simulink model "sm_car"  (R2025a)
settings: Solver=ode23t  StartTime=0.0  StopTime=400  MaxStep=0.4  RelTol=1e-3  AbsTol=1e-3  EnableMultiTasking=on
PreLoadFcn:
  | % Due to usability issue in Repeating Sequence block
  | warning('off','Simulink:Masking:Invalid');
  | 
  | % Eliminate unnecessary warnings in inactive variants
  | % Warnings generated only if you click through inactive variant
  | warning('off','MATLAB:nonExistentField');
  | warning('off','Simulink:Parameters:BlkParamUndefined');
PostLoadFcn:
  | set_param([bdroot '/Vehicle'],'popup_trailer','Off')
  | warning('off','sm:sli:setup:compile:LocalSolverNotSupported')
  | %sm_car_config_maneuver(bdroot,'WOT Braking');
  | sm_car_config_vehicle(bdroot,'false');
  | sm_car_config_logging(bdroot);
InitFcn:
  | sm_car_config_camera;
  | Vehicle = sm_car_vehcfg_checkConfig(Vehicle);
  | sm_car_check_tire_model(bdroot);
StartFcn:
  | tic;
StopFcn:
  | Elapsed_Sim_Time = toc;
  | % disp(['Elapsed Sim Time = ' num2str(Elapsed_Sim_Time)]);
undefined symbols (not defined in the file): Axle1D, AxleIn, Camera, Control, Driver, Free, Init, Maneuver, Pedal, RaceFix, RaceSpin, Scene, ShaftL1, ShaftL2, ShaftR1, ShaftR2, Soft, Stiff, Visual, X, xy_data_car_side, Y, Z
libraries: sm_lib x1546, nesl_utility x528, fl_lib x480, SimscapeFluids_lib x61, sdl_lib x49, simulink x29, ee_lib x7, simulink_extras x6, Linkage_Systems x4, Tire_1x2x x4, AntiRollBar_Systems x2, Linkage_Decoupled x2
(part 79 of 79)

== matlab function sm_car/Driver/Closed Loop/Driver/Lateral Driver/Stanley/Stanley Driver ==
  data: referencePose input; steeringAngle output; currentPose input; v_x input; direction input; L_AXLE_DIST input; MAX_STEERING_ANGLE_DEG input; K_cte_forward input; K_cte_reverse input
function steeringAngle = lateralDrivingController(referencePose, currentPose, v_x, direction, L_AXLE_DIST, MAX_STEERING_ANGLE_DEG, K_cte_forward, K_cte_reverse)
%#codegen % Directive for MATLAB Coder

% lateralDrivingController Implements Stanley method for lateral control.
% Supports forward and reverse driving.
% Based on Hoffmann et al. (2007), "Autonomous Automobile Trajectory Tracking for Off-Road Driving"
%
% Inputs:
%   referencePose: [x_ref, y_ref, yaw_ref] (1x3 double vector)
%       x_ref: Reference x-coordinate (m) on the path (closest point)
%       y_ref: Reference y-coordinate (m) on the path (closest point)
%       yaw_ref: Reference yaw angle (rad) of the path tangent at (x_ref, y_ref)
%   currentPose: [x_curr, y_curr, yaw_curr] (1x3 double vector)
%       x_curr: Current x-coordinate (m) of the vehicle's reference point (e.g., rear axle center)
%       y_curr: Current y-coordinate (m) of the vehicle's reference point
%       yaw_curr: Current yaw angle (rad) of the vehicle
%   v_x: Current longitudinal velocity (m/s) of the vehicle.
%        Positive for forward, can be negative for reverse (though 'direction' input is primary).
%   direction: Driving direction (+1 for forward, -1 for reverse). (scalar double)
%
% Output:
%   steeringAngle: Calculated steering angle (rad) of the front wheels.
%                  Positive for left turn, negative for right turn.

% --- Controller Parameters (Tunable) ---
% K_cte = Driver.Lateral.NForward.Value  ;  % Cross-track error gain (Stanley gain 'k'). Adjust based on vehicle.
              % Typical values: 0.3 to 1.0. Higher values lead to more aggressive correction.

% L_AXLE_DIST = Driver.Lateral.xWheelbase.Value; % Distance from the vehicle's reference point (currentPose)
                                                % to the front axle (m). If currentPose is rear axle, this is wheelbase.

SOFTENING_CONSTANT_V = 0.1; % Small constant (epsilon) to prevent division by zero or
                            % overly aggressive steering at very low speeds (m/s).
                            % Should be small, e.g., 0.01 to 0.5.

MAX_STEERING_ANGLE = MAX_STEERING_ANGLE_DEG * (pi/180)  ; % Maximum steering angle (radians)
% MIN_VELOCITY_FOR_CONTROL is implicitly handled by SOFTENING_CONSTANT_V and using abs(v_x)

% --- Input Validation / Pre-processing (Basic) ---
referencePose = referencePose(:)';
currentPose = currentPose(:)';

% --- Extract Pose Components ---
x_vehicle_ref_pt   = currentPose(1); % x of vehicle's defined reference point (e.g., rear axle)
y_vehicle_ref_pt   = currentPose(2); % y of vehicle's defined reference point
yaw_vehicle        = currentPose(3); % Vehicle's current yaw angle

x_path   = referencePose(1); % x of closest point on path
y_path   = referencePose(2); % y of closest point on path
yaw_path = referencePose(3); % Tangent angle of path at (x_path, y_path)

% --- 1. Calculate Front Axle Position ---
% Stanley controller operates on the error at the front axle.
% (x_fa, y_fa) in the paper's notation.
x_front_axle = x_vehicle_ref_pt + L_AXLE_DIST * cos(yaw_vehicle);
y_front_axle = y_vehicle_ref_pt + L_AXLE_DIST * sin(yaw_vehicle);

% --- 2. Calculate Heading Error (phi_e in paper, psi_e here) ---
% Difference between path yaw and vehicle yaw.
% phi_e = yaw_path - yaw_vehicle
heading_error_raw = yaw_path - yaw_vehicle;
psi_e = atan2(sin(heading_error_raw), cos(heading_error_raw)); % Normalize to [-pi, pi]

% --- 3. Calculate Cross-Track Error (e_fa) at the Front Axle ---
% As per Hoffmann et al. (2007), e_fa is positive if the path is to the
% RIGHT of the vehicle's front axle.
% e_fa = (x_front_axle - x_path) * sin(yaw_path) - (y_front_axle - y_path) * cos(yaw_path);
%
% Let dx_fa = x_front_axle - x_path
% Let dy_fa = y_front_axle - y_path
% The vector from path point to front axle is [dx_fa, dy_fa].
% The path tangent vector is [cos(yaw_path), sin(yaw_path)].
% The path normal vector pointing to the RIGHT of the path is [sin(yaw_path), -cos(yaw_path)].
% e_fa is the projection of [dx_fa, dy_fa] onto this normal vector.
dx_fa = x_front_axle - x_path;
dy_fa = y_front_axle - y_path;

e_fa = dx_fa * sin(yaw_path) - dy_fa * cos(yaw_path);
% Note on sign:
% If front axle is to the LEFT of path, e_fa will be NEGATIVE.
% If front axle is to the RIGHT of path, e_fa will be POSITIVE.

% --- 4. Calculate Steering Angle Components ---

% Cross-track error steering component (delta_e in paper's combined formula)
% delta_e = arctan(k * e_fa / (v_x + softening_constant))
% Use absolute velocity for the denominator to handle forward/reverse consistently
% and add softening constant.
% The paper's v_x in the denominator implies speed magnitude.
effective_velocity_for_atan = abs(v_x) + SOFTENING_CONSTANT_V;

if direction == 1
    delta_cte = atan2(K_cte_forward *  e_fa, effective_velocity_for_atan);
else % if direction == -1
    delta_cte = atan2(K_cte_reverse * -e_fa, effective_velocity_for_atan);
end

% --- 5. Combine Steering Components (Stanley Law) with Directionality ---
% Standard Stanley Law for forward motion:
% steeringAngleUnsaturated = psi_e + delta_cte;
%
% For REVERSE motion (direction = -1):
% The overall steering command needs to be inverted because the vehicle steers
% from the "rear" effectively.
%   - If heading error (psi_e) is positive (path to the left of vehicle yaw),
%     for forward, steer left. For reverse, to make rear go left, steer front right.
%   - If cross-track error (e_fa negative -> front axle left of path),
%     for forward, delta_cte is negative (steer right). For reverse, to make
%     front axle move right (and thus vehicle move right towards path), steer front left.
%
% So, the entire calculated "forward" steering command is multiplied by 'direction'.
steeringAngleUnsaturated = direction * (psi_e + delta_cte);

% --- 6. Saturate Steering Angle ---
if steeringAngleUnsaturated > MAX_STEERING_ANGLE
    steeringAngle = MAX_STEERING_ANGLE;
elseif steeringAngleUnsaturated < -MAX_STEERING_ANGLE
    steeringAngle = -MAX_STEERING_ANGLE;
else
    steeringAngle = steeringAngleUnsaturated;
end

% --- (Optional) Debugging Outputs ---
% coder.extrinsic('fprintf'); % Allow fprintf for debugging during simulation
% fprintf('Dir: %d, YawVeh: %.2f, YawPath: %.2f, psi_e: %.2f\n', direction, yaw_vehicle, yaw_path, psi_e);
% fprintf('x_fa: %.2f, y_fa: %.2f, e_fa: %.2f\n', x_front_axle, y_front_axle, e_fa);
% fprintf('v_x: %.2f, eff_v: %.2f, delta_cte: %.2f\n', v_x, effective_velocity_for_atan, delta_cte);
% fprintf('UnsatSteer: %.3f, Steering cmd: %.3f\n', steeringAngleUnsaturated, steeringAngle);

end

== matlab function sm_car/Driver/Closed Loop/Driver/Longitudinal Driver/Longitudinal Driver ==
  settings: sampleTime=0.1
  data: pp_preview_dist_pts input; AccelCmd output; pp_preview_speed_pts input; ad_vehicle input; current_vx input; dir input; current_slope_rad input; SPEED_LOOKAHEAD_TIME input; VEHICLE_MASS_KG input; GRAVITY_MPS2 input; C_ROLLING_RESISTANCE_COEFF input; C_AERO_DRAG_COEFF input; MAX_NET_DRIVING_FORCE_N input; MAX_NET_BRAKING_FORCE_N input; KP_SPEED input; KI_SPEED input; MAX_ACCEL_MPS2 input; MAX_DECEL_MPS2 input; integral_error_input input; DecelCmd output; v_error_out output
function [AccelCmd, DecelCmd, v_error_out] = longitudinalSpeedController(...
    pp_preview_dist_pts, ...     % Preview segment: cumulative distances (m)
    pp_preview_speed_pts, ...    % Preview segment: target speeds (m/s)
    ad_vehicle, ...              % Current distance of vehicle along path (m)
    current_vx, ...              % Vehicle's current longitudinal velocity (m/s)
    dir, current_slope_rad, ...       % Current road slope/gradient (radians, positive for uphill)    
    SPEED_LOOKAHEAD_TIME, ...    % Lookahead time (s)
    VEHICLE_MASS_KG, ...         % Vehicle mass (kg)
    GRAVITY_MPS2, ...            % Acceleration due to gravity (m/s^2)
    C_ROLLING_RESISTANCE_COEFF, ...    % Rolling resistance coefficient
    C_AERO_DRAG_COEFF, ...             % Aerodynamic drag coefficient (0.5 * rho * A * Cd)
    MAX_NET_DRIVING_FORCE_N, ... % Max net driving force at wheels (engine limit - min resistances)
    MAX_NET_BRAKING_FORCE_N, ... % Max net braking force at wheels (brake limit + engine braking if modeled)
    KP_SPEED, ...                % Proportional gain for speed PI controller (normalized value using max_force_contribution)
    KI_SPEED, ...                % Integral gain for speed PI controller (normalized value using max_force_contribution)
    MAX_ACCEL_MPS2, ...          % Max desired acceleration (for feedforward and limiting)
    MAX_DECEL_MPS2, ...          % Max desired deceleration (negative value, e.g., -5 m/s^2)
    integral_error_input)...     % Externally integrated speed error (m) %#ok<INUSD>

%#codegen

% longitudinalSpeedController Implements a PI controller with feedforward
% for velocity tracking, outputting acceleration/deceleration commands and speed error.
% Designed for continuous-time simulation with external error integration.
%
% Outputs:
%   AccelCmd: Normalized acceleration command [0, 1]
%   DecelCmd: Normalized deceleration command [0, 1] (positive value)
%   v_error_out: Current speed error (v_target - v_actual) (m/s)

%  1. Determine Target Velocity and Desired Acceleration from Preview 
lookahead_dist_for_speed = current_vx * SPEED_LOOKAHEAD_TIME;
target_cumulative_dist_for_speed = ad_vehicle + lookahead_dist_for_speed;

num_preview_pts = length(pp_preview_dist_pts);
v_target_at_lookahead = current_vx; % Default to current speed if no preview

thisSeg = 0;
pp_preview_speed_pts = pp_preview_speed_pts*dir;
if num_preview_pts > 0
    if target_cumulative_dist_for_speed <= pp_preview_dist_pts(1)
        v_target_at_lookahead = pp_preview_speed_pts(1);
    elseif target_cumulative_dist_for_speed >= pp_preview_dist_pts(end)
        v_target_at_lookahead = pp_preview_speed_pts(end);
    else
        % Interpolate to find target speed at lookahead distance
        % (Using existing interpolation logic, could be replaced with interp1)
        for n = 1:(num_preview_pts-1)
            if target_cumulative_dist_for_speed >= pp_preview_dist_pts(n) && ...
               target_cumulative_dist_for_speed < pp_preview_dist_pts(n+1)
                % Ensure denominator is not zero for robust interpolation
                fraction_denom = pp_preview_dist_pts(n+1) - pp_preview_dist_pts(n);
                if fraction_denom > 1e-6 % Avoid division by zero if points are coincident
                    fraction = (target_cumulative_dist_for_speed - pp_preview_dist_pts(n)) / fraction_denom;
                    v_target_at_lookahead = pp_preview_speed_pts(n) + ...
                                       fraction * (pp_preview_speed_pts(n+1) - pp_preview_speed_pts(n));
                else % Points are too close, take the speed of the first point of the pair
                    v_target_at_lookahead = pp_preview_speed_pts(n);
                end
                break; 
            end
            thisSeg = n;
        end
         % Handle case where loop finishes, and target is beyond the last segment start but not caught by pp_preview_dist_pts(end)
         if (thisSeg == (num_preview_pts-1)) && (target_cumulative_dist_for_speed >= pp_preview_dist_pts(end))
            v_target_at_lookahead = pp_preview_speed_pts(end);
         end
    end
end

% Determine desired feedforward acceleration based on a short lookahead on the preview path
idx_current_on_preview = 1;
for n = 1:num_preview_pts
    if ad_vehicle >= pp_preview_dist_pts(n)
        idx_current_on_preview = n;
    else
        break;
    end
end

idx_future_on_preview = idx_current_on_preview;
dist_for_accel_calc = current_vx * 0.1; % Short distance ahead for accel calculation (e.g., 0.2s at current speed)
for n = idx_current_on_preview:num_preview_pts
    if (pp_preview_dist_pts(n) - ad_vehicle) >= dist_for_accel_calc
        idx_future_on_preview = n;
        break;
    end
    if n == num_preview_pts % Reached end of preview
        idx_future_on_preview = num_preview_pts;
    end
end

a_desired_feedforward = 0.0; % Initialize
if idx_future_on_preview > idx_current_on_preview && num_preview_pts > 1
    delta_v = pp_preview_speed_pts(idx_future_on_preview) - pp_preview_speed_pts(idx_current_on_preview);
    delta_d = pp_preview_dist_pts(idx_future_on_preview) - pp_preview_dist_pts(idx_current_on_preview);

    if delta_d > 1e-3 % Ensure segment has some physical length
        v_avg_segment = (pp_preview_speed_pts(idx_future_on_preview) + pp_preview_speed_pts(idx_current_on_preview)) / 2.0;
        
        denominator_v_avg = max(0.1, abs(v_avg_segment)); % Robust denominator for delta_t
        delta_t_segment = delta_d / denominator_v_avg;

        MIN_SEGMENT_TIME_FOR_FF = 1e-3; % Min segment time (s) for a meaningful FF accel calculation
        if delta_t_segment > MIN_SEGMENT_TIME_FOR_FF
            a_desired_feedforward = delta_v / delta_t_segment;
        end
    end
end

if(dir>0)
a_desired_feedforward = max(MAX_DECEL_MPS2, min(a_desired_feedforward, MAX_ACCEL_MPS2)); % Clamp
else
a_desired_feedforward = max(-MAX_ACCEL_MPS2, min(a_desired_feedforward, -MAX_DECEL_MPS2)); % Clamp
end


%  2. Calculate Feedforward Force using Simple Vehicle Model 
F_rolling = C_ROLLING_RESISTANCE_COEFF * VEHICLE_MASS_KG * GRAVITY_MPS2 * cos(current_slope_rad);
F_aero    = C_AERO_DRAG_COEFF * current_vx^2;
F_gravity = VEHICLE_MASS_KG * GRAVITY_MPS2 * sin(current_slope_rad);
F_resist = F_rolling + F_aero + F_gravity;
F_wheels_feedforward = VEHICLE_MASS_KG * a_desired_feedforward - F_resist;

%  3. PI Feedback Controller 
v_error = v_target_at_lookahead - current_vx;
P_term = KP_SPEED * v_error;

% I_term uses externally integrated error
I_term_unclamped = KI_SPEED * integral_error_input;

% Anti-windup: Clamp the force contribution of the I-term
% This assumes integral_error_input is the raw integral.
% The clamping limits the *effect* of very large integrated errors.
max_force_contribution = max(MAX_NET_DRIVING_FORCE_N, MAX_NET_BRAKING_FORCE_N);
I_term = max(-max_force_contribution, min(I_term_unclamped, max_force_contribution));

% Change the PI control to physical values
F_pi_correction = max_force_contribution * (P_term + I_term);

%  4. Combine Feedforward and Feedback 
F_total_desired_at_wheels = F_wheels_feedforward + F_pi_correction;

%  5. Convert Total Desired Force to Normalized Actuation Command [-1, +1] 
actuationCmd = 0.0; % This is the command before any (external) rate limiting

if F_total_desired_at_wheels > 0 % Needs net driving force
    if MAX_NET_DRIVING_FORCE_N > 1e-6 
        actuationCmd = F_total_desired_at_wheels / MAX_NET_DRIVING_FORCE_N;
    end
    actuationCmd = max(0, min(actuationCmd, 1.0)); % Clamp to [0, 1]

elseif F_total_desired_at_wheels < 0 % Needs net braking force
    if MAX_NET_BRAKING_FORCE_N > 1e-6
        actuationCmd = F_total_desired_at_wheels / MAX_NET_BRAKING_FORCE_N; % Will be negative
    end
    actuationCmd = max(-1.0, min(actuationCmd, 0)); % Clamp to [-1, 0]
else
    actuationCmd = 0.0; % Coast
end

% Ensure strictly within [-1, 1] (already handled by clamping in step 5)
% actuationCmd = max(-1.0, min(actuationCmd, 1.0));

% Outputs
if actuationCmd >= 0
    AccelCmd = actuationCmd;
    DecelCmd = 0.0;
else
    AccelCmd = 0.0;
    DecelCmd = -actuationCmd; % DecelCmd is positive, range [0, 1]
end

v_error_out = v_error; % Output current speed error for external integration

%  Debugging Outputs (Optional, ensure coder.extrinsic if used in codegen)
% coder.extrinsic('fprintf');
% fprintf('Vcurr: %.2f, Vtgt_LH: %.2f, Verr: %.2f\n', current_vx, v_target_at_lookahead, v_error);
% fprintf('Ades_FF: %.2f, F_wheels_FF: %.1f, F_PI: %.1f, F_total_des: %.1f\n', ...
%         a_desired_feedforward, F_wheels_feedforward, F_pi_correction, F_total_desired_at_wheels);
% fprintf('CmdUnrated: %.3f\n', actuationCmd);

end

== matlab function sm_car/Driver/Closed Loop/Maneuver/MATLAB Function ==
  data: ref_z output; ad output; ref_x output; ref_y output; ref_ayaw output; vTarget output; ld output; cp output; simres output; pp_preview_x_pts output; pp_preview_y_pts output; pp_preview_yaw_pts output; pp_preview_dist_pts output; pp_preview_speed_pts output; idx_ptMin output; p input; q input; posx input; posy input; posz input; speed input; xywin input; yaw input; dist input; pd input; maxld input; minSpd input; speedGain input; idx_ptMin_prev input; nPreviewPoints parameter
function [ref_z,ad,ref_x,ref_y,ref_ayaw,vTarget,ld,cp,  simres, ...
          pp_preview_x_pts, pp_preview_y_pts, pp_preview_yaw_pts, pp_preview_dist_pts, pp_preview_speed_pts,idx_ptMin] = ...
          getPoseCurRef(p,q,posx,posy,posz,speed,xywin,yaw,dist,pd, ...
                        maxld, minSpd, speedGain, idx_ptMin_prev, nPreviewPoints)

% This function determines the target pose for the vehicle.  It
% interpolates within the provided trajectory to determine the target
% x-y position, yaw angle, and speed. The targets are defined with respect
% to distance along the target trajectory.  The first portion of the
% function determines the distance along the trajectory that the vehicle
% has traveled (ad).  Once that is found, the function interpolates to find
% the target pose at the preview distance (ad+pd).

npts = length(posx);

% Look for nearest point in a window near last evaluation
% Obtain window
if (idx_ptMin_prev == -1)
    % For first evaluation, use entire list of points
    ptlist = 1:npts;
elseif((idx_ptMin_prev-xywin)<1)
    % Window overlaps at lower end: take points from upper end
    win2 = (npts+idx_ptMin_prev-xywin):1:npts;
    win1 = 1:(idx_ptMin_prev+xywin);
    ptlist = [win1 win2];
elseif((idx_ptMin_prev+xywin)>npts)
    % Window overlaps at upper end: take points from lower end
    win2 = (idx_ptMin_prev-xywin):1:npts;
    win1 = 1:(idx_ptMin_prev+xywin-npts);
    ptlist = [win1 win2];
else
    % No overlap: use window
    ptlist = (idx_ptMin_prev-xywin):1:(idx_ptMin_prev+xywin);
end

% Find closest supplied trajectory point to current car position
distances = hypot(p(1) - posx,p(2) - posy);
distances_srch = distances(ptlist);
[~, idx_ptlist] = min(distances_srch);
idx_ptMin = ptlist(idx_ptlist);

%% Identify two trajectory points ahead of and behind closest supplied point
% A, B, C (closest), D, E
idx_ptC = idx_ptMin;
idx_ptA = idx_ptMin-2;
idx_ptB = idx_ptMin-1;
idx_ptD = idx_ptMin+1;
idx_ptE = idx_ptMin+2;

% If we are at end of trajectory, wrap point index
if (idx_ptA<=0),   idx_ptA = idx_ptA+npts; end
if (idx_ptB<=0),   idx_ptB = idx_ptB+npts; end
if (idx_ptD>npts), idx_ptD = idx_ptD-npts; end
if (idx_ptE>npts), idx_ptE = idx_ptE-npts; end

% Extract trajectory point x-y locations
ptA = [posx(idx_ptA); posy(idx_ptA)];
ptB = [posx(idx_ptB); posy(idx_ptB)];
ptC = [posx(idx_ptC); posy(idx_ptC)];
ptD = [posx(idx_ptD); posy(idx_ptD)];
ptE = [posx(idx_ptE); posy(idx_ptE)];

%% Find line separating trajectory segments BC, CD
% Find angle of line connecting BD
qBD = atan2(ptD(2)-ptB(2),ptD(1)-ptB(1));

% Angle of line separating BC, CD is normal to that line
qC  = qBD+pi/2;

%% Determine if we are nearest to trajectory segment BC or BD
% Check if vehicle location and point B on same side of line
% separating segments BC and BD
segBC = arePointsOnSameSide(ptC(1), ptC(2), tan(qC), p(1), p(2), ptB(1), ptB(2));

%% Find vehicle line segment 
% Segment is parallel to closest trajectory segment on which vehicle lies
if(segBC)
   % Use segment BC
   % Line dividing segments AB and BC is normal to line AC 
   qR = atan2(ptC(2)-ptA(2),ptC(1)-ptA(1))+pi/2;
   % Line dividing segments BC and CD has already been found 
   qF = qC;

   ptR = ptB;  % Rear point of segment is point B
   ptF = ptC;  % Front point of segment is point C

   % Angle of vehicle line segment is same as angle of segment BC
   qV = atan2(ptC(2)-ptB(2),ptC(1)-ptB(1));
    % Distance along trajectory to rear of segment
   distR    = dist(idx_ptB);
else
   % Use segment CD
   % Line dividing segments BC and CD has already been found 
   qR = qC;
   % Line dividing segments CD and DE is normal to line CE 
   qF = atan2(ptE(2)-ptC(2),ptE(1)-ptC(1))+pi/2;

   ptR = ptC;    % Rear point of segment is point B
   ptF = ptD;    % Front point of segment is point C

   % Angle of vehicle line segment is same as angle of segment CD
   qV = atan2(ptD(2)-ptC(2),ptD(1)-ptC(1));
    % Distance along trajectory to rear of segment
   distR = dist(idx_ptC);
end

% Length of trajectory segment
distSeg  = sqrt((ptF(1)-ptR(1))^2+(ptF(2)-ptR(2))^2);

% Find endpoints of vehicle line segment
[xR, yR] = findIntersection(p(1), p(2), tan(qV), ptR(1), ptR(2), tan(qR));
[xF, yF] = findIntersection(p(1), p(2), tan(qV), ptF(1), ptF(2), tan(qF));

% Length of vehicle line segment
distFR = sqrt((xR-xF)^2+(yR-yF)^2);

% Distance of vehicle location from rear of vehicle line segment
% Handle potential division by zero if distFR is very small (e.g. vehicle exactly on ptR or ptF)
if distFR < 1e-6 
    distvR = 0;
else
    distvR = sqrt((xR-p(1))^2+(yR-p(2))^2);
end

% Percentage of distance from vehicle to rear of vehicle line segment 
% Do not permit percentage to go above 100%
% Occurs when vehicle is far from line on inside of curve
segPcnt = min(distvR/distFR,1);

% Distance along trajectory = 
%   Distance to rear of trajectory segment + 
%   length of closest trajectory segment * 
%   percent of vehicle line segment already completed
ad = distR+segPcnt*distSeg;

% Find angle between vehicle location, forward point, and track trajectory
vec_F2v  = ptF - [p(1); p(2)];
vec_F2R  = ptF - ptR;

% Use cosine formula to obtain angle
cos_ang_new = dot(vec_F2v,vec_F2R)/(norm(vec_F2v)*norm(vec_F2R) + eps); % Add eps for stability

% Bound cosine of angle between eps and 1
cos_ang_new = max(cos_ang_new,eps);
cos_ang_new = min(cos_ang_new,1-eps);

% Use angle to obtain lateral distance of vehicle from trajectory
ld = norm(vec_F2v)*sin(acos(cos_ang_new));

%  Prepare interpolation data (handles wrapping) 
% Ensure dist is monotonically increasing for interp1
if any(diff(dist) <= 0) && npts > 1
    % This case should ideally not happen with well-formed 'dist' arrays.
    % If it does, it indicates an issue with the input trajectory 'dist'.
    % For robustness, one might try to fix it or error out.
    % Here, we'll assume 'dist' is mostly fine and proceed,
    % but interp1 might behave unexpectedly.
    % A simple fix for non-codegen mode could be to use unique:
    % [dist_unique, ia, ~] = unique(dist);
    % posx_unique = posx(ia); ... etc.
    % But this is complex for codegen.
    % The provided dist4interp tries to handle wrapping, which is the main concern.
end

% Pose targets for Stanley controller (distance cumulatively sums)
if npts > 1
    dist4interp = [-dist(end)+dist(1:end-1); dist; dist(end)+dist(2:end)];
    posx4interp = [           posx(1:end-1); posx;           posx(2:end)];
    posy4interp = [           posy(1:end-1); posy;           posy(2:end)];
    posz4interp = [           posz(1:end-1); posz;           posz(2:end)];
    speed4interp= [          speed(1:end-1);speed;          speed(2:end)];
    % Wrap the interpolation vector for yaw.
    % Necessary to avoid obtaining values between yaw(end) and yaw(1)
    yaw4interp  = [-(yaw(end)-yaw(1)) + yaw(1:end-1);  yaw;  (yaw(end)-yaw(1))+ yaw(2:end)];
else % Single point trajectory
    dist4interp = dist;
    posx4interp = posx;
    posy4interp = posy;
    posz4interp = posz;
    speed4interp = speed;
    yaw4interp = yaw;
end

%  Current vehicle pose output 
cp = [p(1);p(2);q(3)*180/pi]'; % q(3) is vehicle yaw in rad, convert to deg for cp

% Reference point obtained from supplied trajectory
% Interpolate using Actual distance (ad) + preview distance (pd)
target_dist_single_ref = ad + pd;
ref_x    = interp1(dist4interp,posx4interp,target_dist_single_ref,'pchip');
ref_y    = interp1(dist4interp,posy4interp,target_dist_single_ref,'pchip');
ref_ayaw = interp1(dist4interp,yaw4interp, target_dist_single_ref,'pchip');
ref_z    = interp1(dist4interp,posz4interp,target_dist_single_ref,'pchip'); % For visualization

% Handle NaNs from interp1 if target_dist_single_ref is outside bounds
% (though wrapped dist4interp should prevent this for cyclic paths if pd is reasonable)
if isnan(ref_x); ref_x = posx(idx_ptMin); end % Fallback to closest raw point
if isnan(ref_y); ref_y = posy(idx_ptMin); end
if isnan(ref_ayaw); ref_ayaw = yaw(idx_ptMin); end
if isnan(ref_z); ref_z = posz(idx_ptMin); end

% Reference velocity obtained from supplied trajectory
% Interpolate using actual distance 
vx_cp_trajectory = interp1(dist4interp,speed4interp,ad);
if isnan(vx_cp_trajectory); vx_cp_trajectory = speed(idx_ptMin); end

% Protect for NaNs
ref_x(isnan(ref_x)) = 0;
ref_y(isnan(ref_y)) = 0;
ref_ayaw(isnan(ref_ayaw)) = 0;
ref_z(isnan(ref_z)) = 0;

% Scale speed target
% Reduce speed target if car is far from the target trajectory
if ld < maxld
    % If near target path, use target speed
    vTarget = vx_cp_trajectory * speedGain;
else
    % If too far off track, drop to slow target speed
    vTarget = sign(vx_cp_trajectory) * minSpd;
end

%  Generate Preview Path Segment for Pure Pursuit 
% The segment will span from 'ad' to 'ad + pd'
% 'pd' input now also defines the length of this preview segment
pp_preview_dist_pts = ad + linspace(0, pd, nPreviewPoints);

% Interpolate to get x, y, yaw for these preview points
pp_preview_x_pts     = interp1(dist4interp, posx4interp, pp_preview_dist_pts, 'pchip');
pp_preview_y_pts     = interp1(dist4interp, posy4interp, pp_preview_dist_pts, 'pchip');
pp_preview_yaw_pts   = interp1(dist4interp, yaw4interp, pp_preview_dist_pts, 'pchip');
pp_preview_speed_pts = interp1(dist4interp, speed4interp, pp_preview_dist_pts, 'pchip'); % Added for vx

% Handle potential NaNs from interpolation (e.g., if pd is too large and goes off-path)
% A simple strategy: fill with the last valid point of the original trajectory or the closest point.
% For robustness, we use the values at idx_ptMin if NaNs occur.
for i = 1:nPreviewPoints
    if isnan(pp_preview_x_pts(i)); pp_preview_x_pts(i) = posx(idx_ptMin); end
    if isnan(pp_preview_y_pts(i)); pp_preview_y_pts(i) = posy(idx_ptMin); end
    if isnan(pp_preview_yaw_pts(i)); pp_preview_yaw_pts(i) = yaw(idx_ptMin); end
    if isnan(pp_preview_speed_pts(i)); pp_preview_speed_pts(i) = speed(idx_ptMin); end % Added for vx
    % pp_preview_dist_pts(i) should not be NaN as it's from linspace
end


% Outputs for debugging calculation
simres = [idx_ptA idx_ptB idx_ptC idx_ptD idx_ptE qC segBC segPcnt xR yR  xF yF p(1) p(2) ad distR distSeg];

end

% Helper functions 
% findIntersection and arePointsOnSameSide should be defined as local functions
% or be on the MATLAB path if they are separate .m files. For a single MATLAB Function
% block, they should be local.

function [x_intersect, y_intersect] = findIntersection(x1, y1, m1, x2, y2, m2)
    %#codegen
    % Check if the slopes are equal (parallel lines)
    if abs(m1 - m2) < 1e-9 % Compare with tolerance
        % Handle parallel lines: for codegen, avoid error(), return NaNs or specific values
        x_intersect = NaN;
        y_intersect = NaN;
        % For critical applications, this case needs careful handling based on requirements.
        % One might assert or use a default behavior.
        %coder.varsize('error_msg'); error('Invalid trajectory points. The lines are parallel and do not intersect.');
        return;
    end
    
    % Calculate the intersection point
    x_intersect = (y2 - y1 + m1*x1 - m2*x2) / (m1 - m2);
    y_intersect = m1 * (x_intersect - x1) + y1;
end

function same_side = arePointsOnSameSide(x0, y0, m, x1, y1, x2, y2)
    %#codegen
    % Calculate the line coefficients for line y - y0 = m(x - x0) => mx - y - (mx0 - y0) = 0
    % a*x + b*y + c = 0
    a = m; 
    b = -1;  
    c = -m*x0 + y0; 
    
    % Calculate the line equation value for both points
    value1 = a*x1 + b*y1 + c;
    value2 = a*x2 + b*y2 + c;
    
    % Check if both values have the same sign (or one is zero)
    % Product > 0 means same sign. Product == 0 means one point is on the line.
    same_side = (value1 * value2) >= 0; % Include points on the line as "same side"
end

== matlab function sm_car/Controller/TrqVec 4Motor/Power_TqVec/Torque Vectoring/Calculate Torque Split ==
  data: enable input; max_delta_trq input; max_tq input; tq_l_out output; tq_l input; tq_r input; tq_r_out output; tq_tv input; brk input
function [tq_l_out,tq_r_out] = fcn(enable,max_delta_trq,max_tq,tq_l,tq_r,tq_tv,brk)

% enable: flag to turn on torque vectoring
%         True if steering wheel is turned and non-zero vehicle speed
% brk   : flag to turn on torque vectoring
%         True if not braking


% Limit difference in torque between tires lower of 
% (input parameter) and max/min motor torque
t_lim=min(max_tq-abs(tq_l),max_tq-abs(tq_r));
delta_t=min(max_delta_trq,min(t_lim,abs(tq_tv)))*sign(tq_tv)*enable;

if brk>0 
    % Not braking. Use torque vectoring
    tq_l_out=(tq_l-delta_t)*brk;
    tq_r_out=(tq_r+delta_t)*brk;
else
    % No adjustments due to torque vectoring
    tq_l_out=tq_l;
    tq_r_out=tq_r;
end

== stateflow chart sm_car/Controller/TrqVec 4Motor/Brake Control/ABS/Valve Control L1/Logic ==
  state Inactive
    entry:
    Mod_State = 1;
    Mod_Dur = 10;
  state Initial_Release
    entry:
    Mod_State = 2;
    Mod_Dur = 10;
  state Initial_Apply
    entry:
    Mod_State = 1;
    Mod_Dur = 6;
  state Release
    entry:
    Mod_State = 2;
    Mod_Dur = 6;
  state Apply
    entry:
    Mod_State = 1;
    Mod_Dur = 2;
  state Hold
    entry:
    Mod_State = 0;
    Mod_Dur = 6;
  (default) -> Inactive
  Apply -> Inactive [order 2] : [vSpdEst <0.1]
  Release -> Inactive [order 2] : [vSpdEst <0.1]
  Inactive -> Initial_Release : [Slip>0.5]
  Initial_Release -> Initial_Apply : [Slip<0.1]
  Release -> Initial_Apply [order 1] : [Slip <0.05]
  Initial_Apply -> Hold [order 2] : [Slip>0.1]
  Initial_Apply -> Apply [order 1] : [after(10,msec)]
  Hold -> Release [order 2] : [Slip > 0.25]
  Hold -> Apply [order 1] : [after(40,msec)]
  Apply -> Hold [order 1] : [Slip > 0.1]
  data: Slip input; Mod_State output; Mod_Dur output; vSpdEst input

== stateflow chart sm_car/Controller/TrqVec 4Motor/Brake Control/ABS/Valve Control L2/Logic ==
  state Inactive
    entry:
    Mod_State = 1;
    Mod_Dur = 10;
  state Initial_Release
    entry:
    Mod_State = 2;
    Mod_Dur = 10;
  state Initial_Apply
    entry:
    Mod_State = 1;
    Mod_Dur = 6;
  state Release
    entry:
    Mod_State = 2;
    Mod_Dur = 6;
  state Apply
    entry:
    Mod_State = 1;
    Mod_Dur = 2;
  state Hold
    entry:
    Mod_State = 0;
    Mod_Dur = 6;
  (default) -> Inactive
  Apply -> Inactive [order 2] : [vSpdEst <0.1]
  Release -> Inactive [order 2] : [vSpdEst <0.1]
  Inactive -> Initial_Release : [Slip>0.5]
  Initial_Release -> Initial_Apply : [Slip<0.1]
  Release -> Initial_Apply [order 1] : [Slip <0.05]
  Initial_Apply -> Hold [order 2] : [Slip>0.1]
  Initial_Apply -> Apply [order 1] : [after(10,msec)]
  Hold -> Release [order 2] : [Slip > 0.25]
  Hold -> Apply [order 1] : [after(40,msec)]
  Apply -> Hold [order 1] : [Slip > 0.1]
  data: Slip input; Mod_State output; Mod_Dur output; vSpdEst input
